simulink model "DeadtimeTest"  (R2026b)
settings: Solver=ode4  StopTime=fixtureCfg.Duration  FixedStep=experimentCfg.Step
PostLoadFcn:
  | addpath(fullfile(fileparts(fileparts(fileparts(fileparts(fileparts(get_param(bdroot,'FileName')))))),'docs','scripts'));initialize_motor_paths();initialize_motor_model(bdroot);
model workspace (MAT data in the model file):
  currentCfg.Ts = 0.0001
  currentCfg.BandwidthHz = 500
  currentCfg.Kpd = 3.14159265359
  currentCfg.Kpq = 3.76991118431
  currentCfg.Kid = 1570.79632679
  currentCfg.Kiq = 1570.79632679
  currentCfg.Kaw = 1000
  deadtimeCfg.DeadTime = 2e-06
  deadtimeCfg.DeviceDrop = 0
  deadtimeCfg.CurrentBlend = 0.1
  deadtimeCfg.ModelEnable = 1
  deadtimeCfg.CompensationEnable = 1
  deadtimeCfg.CompensationScale = 1
  deadtimeCfg.SwitchingStep = 1e-07
  experimentCfg.Step = 5e-06
  experimentCfg.LogTs = 0.0001
  experimentCfg.Duration = 1.5
  experimentCfg.Mode = 2
  experimentCfg.UseInverter = 1
  experimentCfg.UseTiming = 1
  experimentCfg.UseMechanical = 1
  experimentCfg.ImposedElectricalSpeed = 0
  experimentCfg.IdReference = 0
  experimentCfg.IqReference = 2
  experimentCfg.IqInitial = 0
  experimentCfg.SpeedReference = 40
  experimentCfg.SpeedInitial = 0
  experimentCfg.PositionReference = 1
  experimentCfg.PositionInitial = 0
  experimentCfg.CommandTime = 0.05
  experimentCfg.LoadTorque = 0.1
  experimentCfg.LoadTime = 0.35
  experimentCfg.Enable = 1
  experimentCfg.Reset = 0
  feedforwardCfg.Enable = 0
  feedforwardCfg.ParameterScale = 1
  fixtureCfg.Ts = 0.0001
  fixtureCfg.Duration = 0.03
  fixtureCfg.SolverStep = 5e-06
  fixtureCfg.CurrentAmplitude = 3
  fixtureCfg.FrequencyHz = 50
  fixtureCfg.InitialPhase = 0
  fixtureCfg.ModelEnable = 1
  fixtureCfg.CompensationEnable = 1
  fixtureCfg.Inputs = [3 2.9985196811 2.99408018528 2.98668589381 2.97634410394 2.96306502179 2.94686175219 2.92775028582 2.90574948339 2.88088105703 2.85316954889 2.82264230686 ... (903 elements, 301x3)]
  inverterCfg.Vdc = 48
  inverterCfg.MinDuty = 0.02
  inverterCfg.PwmTs = 0.0001
  inverterCfg.LinearLimit = 26.6043004043
  motionCfg.Ts = 0.001
  motionCfg.NaturalFrequency = 20
  motionCfg.Damping = 0.9
  motionCfg.Kt = 0.21
  motionCfg.Kp = 0.0852380952381
  motionCfg.Ki = 0.952380952381
  motionCfg.Kaw = 20
  motionCfg.PositionKp = 8
  motionCfg.SpeedLimit = 80
  motionCfg.AccelerationLimit = 200
  motionCfg.CurrentLimit = 8
  pmsmCfg.Rs = 0.5
  pmsmCfg.Ld = 0.001
  pmsmCfg.Lq = 0.0012
  pmsmCfg.Flux = 0.035
  pmsmCfg.PolePairs = 4
  pmsmCfg.J = 0.0005
  pmsmCfg.B = 0.0001
  pmsmCfg.Id0 = 0
  pmsmCfg.Iq0 = 0
  pmsmCfg.Speed0 = 0
  pmsmCfg.Position0 = 0
  testStim.time = []
  testStim.signals.values = [3 2.9985196811 2.99408018528 2.98668589381 2.97634410394 2.96306502179 2.94686175219 2.92775028582 2.90574948339 2.88088105703 2.85316954889 2.82264230686 ... (903 elements, 301x3)]
  testStim.signals.dimensions = 3
  timingCfg.Ts = 0.0001
  timingCfg.FeedbackTicks = 1
  timingCfg.ActuationTicks = 1
libraries: Deadtime x2
settings Model: Creator=24322  LastModifiedBy=24322

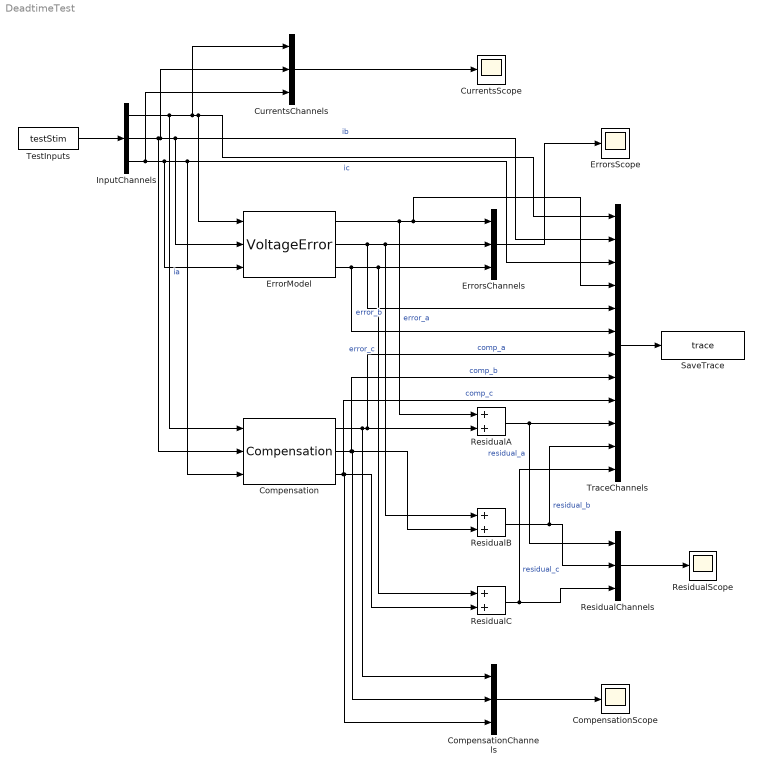
== system DeadtimeTest ==
  Compensation : Deadtime/Compensation  SystemSampleTime=-1  VariantActivationTime=update diagram  EmptyChoice=off  PassThrough=off  PassThroughVariantControl=(default)  EmptyChoiceVariantControl=(default)  AllowFlexibleInterface=on  Latency=0  AutoFrameSizeCalculation=off
  CompensationChannels : Mux  Inputs=3
  CompensationScope : Scope
      settings: Title=Compensation  YLabel=V
  CurrentsChannels : Mux  Inputs=3
  CurrentsScope : Scope
      settings: Title=Currents  YLabel=A
  ErrorModel : Deadtime/VoltageError  SystemSampleTime=-1  VariantActivationTime=update diagram  EmptyChoice=off  PassThrough=off  PassThroughVariantControl=(default)  EmptyChoiceVariantControl=(default)  AllowFlexibleInterface=on  Latency=0  AutoFrameSizeCalculation=off
  ErrorsChannels : Mux  Inputs=3
  ErrorsScope : Scope
      settings: Title=Errors  YLabel=V
  InputChannels : Demux  Outputs=3
  ResidualA : Sum
  ResidualB : Sum
  ResidualC : Sum
  ResidualChannels : Mux  Inputs=3
  ResidualScope : Scope
      settings: Title=Residual  YLabel=V
  SaveTrace : ToWorkspace  VariableName=trace  SaveFormat=Structure With Time  SampleTime=experimentCfg.LogTs
  TestInputs : FromWorkspace  VariableName=testStim  SampleTime=currentCfg.Ts  Interpolate=off  OutputAfterFinalValue=Holding final value
  TraceChannels : Mux  Inputs=12
  wires:
  ResidualChannels/1 -> ResidualScope/1
  CompensationChannels/1 -> CompensationScope/1
  ErrorsChannels/1 -> ErrorsScope/1
  CurrentsChannels/1 -> CurrentsScope/1
  ResidualC/1 -> TraceChannels/12, ResidualChannels/3  "residual_c"
  ResidualB/1 -> TraceChannels/11, ResidualChannels/2  "residual_b"
  ResidualA/1 -> TraceChannels/10, ResidualChannels/1  "residual_a"
  TraceChannels/1 -> SaveTrace/1
  Compensation/3 -> ResidualC/2, CompensationChannels/3, TraceChannels/9  "comp_c"
  ErrorModel/3 -> ResidualC/1, ErrorsChannels/3, TraceChannels/6  "error_c"
  InputChannels/3 -> Compensation/3, TraceChannels/3, ErrorModel/3, CurrentsChannels/3  "ic"
  Compensation/2 -> ResidualB/2, CompensationChannels/2, TraceChannels/8  "comp_b"
  ErrorModel/2 -> ResidualB/1, ErrorsChannels/2, TraceChannels/5  "error_b"
  InputChannels/2 -> ErrorModel/2, TraceChannels/2, CurrentsChannels/2, Compensation/2  "ib"
  Compensation/1 -> ResidualA/2, TraceChannels/7, CompensationChannels/1  "comp_a"
  ErrorModel/1 -> TraceChannels/4, ErrorsChannels/1, ResidualA/1  "error_a"
  InputChannels/1 -> ErrorModel/1, TraceChannels/1, CurrentsChannels/1, Compensation/1  "ia"
  TestInputs/1 -> InputChannels/1
